simulink model "s_c_nbe_m1k"  (R2016b)
settings: Solver=VariableStepAuto  StartTime=0.0  StopTime=1000  RelTol=1e-3  EnableMultiTasking=on
undefined symbols (not defined in the file): Coeffs, fft_stages, n_taps, output_bits, pfb_coeff_gen_calc, xengbits
libraries: xbsIndex_r4 x23639, casper_library_misc x65, casper_library_scopes x4, xbsReplacements_r4 x4, xps_library x3
(part 36 of 198)

== system s_c_nbe_m1k/DDC/dec_fir_async3 ==
  sync_in : Inport
  dv_in : Inport  Port=2
  real1 : Inport  Port=3
  imag1 : Inport  Port=4
  real2 : Inport  Port=5
  imag2 : Inport  Port=6
  real3 : Inport  Port=7
  imag3 : Inport  Port=8
  real4 : Inport  Port=9
  imag4 : Inport  Port=10
  real5 : Inport  Port=11
  imag5 : Inport  Port=12
  real6 : Inport  Port=13
  imag6 : Inport  Port=14
  real7 : Inport  Port=15
  imag7 : Inport  Port=16
  real8 : Inport  Port=17
  imag8 : Inport  Port=18
  real9 : Inport  Port=19
  imag9 : Inport  Port=20
  real10 : Inport  Port=21
  imag10 : Inport  Port=22
  real11 : Inport  Port=23
  imag11 : Inport  Port=24
  real12 : Inport  Port=25
  imag12 : Inport  Port=26
  real13 : Inport  Port=27
  imag13 : Inport  Port=28
  real14 : Inport  Port=29
  imag14 : Inport  Port=30
  real15 : Inport  Port=31
  imag15 : Inport  Port=32
  real16 : Inport  Port=33
  imag16 : Inport  Port=34
  Logical : xbsIndex_r4/Logical  logical_function=OR  inputs=2  en=off  latency=0  precision=Full  arith_type=Unsigned  n_bits=16  bin_pt=0  align_bp=on  dbl_ovrd=off  block_type=logical
  convert_of : Subsystem  AncestorBlock=casper_library_misc/convert_of  mask(convert_of){bit_width_i=44, binary_point_i=34, bit_width_o=18, binary_point_o=17, latency=2, overflow=Saturate, quantization=Round  (unbiased: +/- Inf)}
      mask prompts: bit_width_i "Bit Width In"; binary_point_i "Binary Point In"; bit_width_o "Bit Width Out"; binary_point_o "Binary Point Out"; overflow "Overflow Behaviour"; quantization "Quantization Behaviour"
      mask help:
      | Converts from one 2's complement bit-width
      | and/or binary point position to another.
      | Includes underflow/overflow indicator.
      mask init: same as s_c_nbe_m1k/DDC/dec_fir_async2/convert_of
      settings: AttributesFormatString=[44,34]->[18,17]
      mask TypeOptions overflow: Wrap | Saturate | Error
      mask TypeOptions quantization: Truncate | Round  (unbiased: +/- Inf) | Round  (unbiased: even values)
  convert_of1 : Subsystem  AncestorBlock=casper_library_misc/convert_of  mask(convert_of){bit_width_i=44, binary_point_i=34, bit_width_o=18, binary_point_o=17, latency=2, overflow=Saturate, quantization=Round  (unbiased: +/- Inf)}
      mask prompts: bit_width_i "Bit Width In"; binary_point_i "Binary Point In"; bit_width_o "Bit Width Out"; binary_point_o "Binary Point Out"; overflow "Overflow Behaviour"; quantization "Quantization Behaviour"
      mask help:
      | Converts from one 2's complement bit-width
      | and/or binary point position to another.
      | Includes underflow/overflow indicator.
      mask init: same as s_c_nbe_m1k/DDC/dec_fir_async2/convert_of
      settings: AttributesFormatString=[44,34]->[18,17]
      mask TypeOptions overflow: Wrap | Saturate | Error
      mask TypeOptions quantization: Truncate | Round  (unbiased: +/- Inf) | Round  (unbiased: even values)
  dv_delay : xbsIndex_r4/Delay  rst=off  infoeditControl=Selection of Reset will increase slice count due to use of real FFs and instead of SRLs  en=off  latency=70  reg_retiming=off  dbl_ovrd=off  block_type=delay
      settings: infoedit=Hardware notes: A delay line is a chain, each link of which is an SRL16 or SRL32 followed by a flip-flop.
  fir_col_async1 : Subsystem  AncestorBlock=casper_library_downconverter/fir_col_async  mask(fir_col_async){n_inputs=16, coeff=[-0.0014387  -0.0013164  -0.0011904  -0.0010635 -0.00093843 -0.00081728 -0.00070197   -0.000594 -0.00049456 -0.00040436 -0.00032436 -0.00025272 -0.00019764 -0.00012413  -0.0001761 -3.7164e-05], add_latency=7, mult_latency=7, coeff_bit_width=18, coeff_bin_pt=17, first_stage_hdl=on, adder_imp=DSP48, async=on, bus_input=off, input_width=0, input_bp=0, input_type=Signed, dbl=on}
      mask prompts: n_inputs "Inputs"; coeff "Coefficients"; add_latency "Add latency"; mult_latency "Mult Latency"; coeff_bit_width "Coefficient bit width"; coeff_bin_pt "Coefficient binary point"; first_stage_hdl "Implement first stage of adder trees on output as behavioural HDL"; adder_imp "Adder implementation"; async "Asynchronous ops"; bus_input "Bus input"; input_width "Input bitwidth"; input_bp "Input binary point"; input_type "Input datatype"; dbl "Double col"
      mask init:
      | fir_col_async_init(gcb);
      mask Help: eval('xlWeb(''http://casper.berkeley.edu/wiki/Fir_col'')')
      mask TypeOptions adder_imp: Behavioral | Fabric | DSP48
      mask Callback bus_input:
      | onoff = get_param(gcb, 'bus_input');
      | set_param_state(gcb, 'input_width', onoff)
      | set_param_state(gcb, 'input_bp', onoff)
      | set_param_state(gcb, 'input_type', onoff)
      mask TypeOptions input_type: Signed | Unsigned
  fir_col_async2 : Subsystem  AncestorBlock=casper_library_downconverter/fir_col_async  mask(fir_col_async){n_inputs=16, coeff=[-0.00060248  -0.0008629  -0.0011001  -0.0013106  -0.0014916  -0.0016412  -0.0017585  -0.0018435  -0.0018966  -0.0019194  -0.0019136  -0.0018817  -0.0018267  -0.0017515  -0.0016595  -0.0015541], add_latency=7, mult_latency=7, coeff_bit_width=18, coeff_bin_pt=17, first_stage_hdl=on, adder_imp=DSP48, async=on, bus_input=off, input_width=0, input_bp=0, input_type=Signed, dbl=on}
      mask prompts: n_inputs "Inputs"; coeff "Coefficients"; add_latency "Add latency"; mult_latency "Mult Latency"; coeff_bit_width "Coefficient bit width"; coeff_bin_pt "Coefficient binary point"; first_stage_hdl "Implement first stage of adder trees on output as behavioural HDL"; adder_imp "Adder implementation"; async "Asynchronous ops"; bus_input "Bus input"; input_width "Input bitwidth"; input_bp "Input binary point"; input_type "Input datatype"; dbl "Double col"
      mask init:
      | fir_col_async_init(gcb);
      mask Help: eval('xlWeb(''http://casper.berkeley.edu/wiki/Fir_col'')')
      mask TypeOptions adder_imp: Behavioral | Fabric | DSP48
      mask Callback bus_input:
      | onoff = get_param(gcb, 'bus_input');
      | set_param_state(gcb, 'input_width', onoff)
      | set_param_state(gcb, 'input_bp', onoff)
      | set_param_state(gcb, 'input_type', onoff)
      mask TypeOptions input_type: Signed | Unsigned
  fir_col_async3 : Subsystem  AncestorBlock=casper_library_downconverter/fir_col_async  mask(fir_col_async){n_inputs=16, coeff=[0.0017612   0.0019473    0.002073   0.0021379   0.0021431   0.0020913   0.0019861   0.0018327    0.001637   0.0014057   0.0011457  0.00086469  0.00057007  0.00026925 -3.0764e-05 -0.00032335], add_latency=7, mult_latency=7, coeff_bit_width=18, coeff_bin_pt=17, first_stage_hdl=on, adder_imp=DSP48, async=on, bus_input=off, input_width=0, input_bp=0, input_type=Signed, dbl=on}
      mask prompts: n_inputs "Inputs"; coeff "Coefficients"; add_latency "Add latency"; mult_latency "Mult Latency"; coeff_bit_width "Coefficient bit width"; coeff_bin_pt "Coefficient binary point"; first_stage_hdl "Implement first stage of adder trees on output as behavioural HDL"; adder_imp "Adder implementation"; async "Asynchronous ops"; bus_input "Bus input"; input_width "Input bitwidth"; input_bp "Input binary point"; input_type "Input datatype"; dbl "Double col"
      mask init:
      | fir_col_async_init(gcb);
      mask Help: eval('xlWeb(''http://casper.berkeley.edu/wiki/Fir_col'')')
      mask TypeOptions adder_imp: Behavioral | Fabric | DSP48
      mask Callback bus_input:
      | onoff = get_param(gcb, 'bus_input');
      | set_param_state(gcb, 'input_width', onoff)
      | set_param_state(gcb, 'input_bp', onoff)
      | set_param_state(gcb, 'input_type', onoff)
      mask TypeOptions input_type: Signed | Unsigned
  fir_col_async4 : Subsystem  AncestorBlock=casper_library_downconverter/fir_col_async  mask(fir_col_async){n_inputs=16, coeff=[-0.0034012  -0.0033949  -0.0032965  -0.0031135   -0.002855  -0.0025319  -0.0021562  -0.0017405  -0.0012982 -0.00084229  -0.0003857  5.9318e-05  0.00048145  0.00087067   0.0012182   0.0015169], add_latency=7, mult_latency=7, coeff_bit_width=18, coeff_bin_pt=17, first_stage_hdl=on, adder_imp=DSP48, async=on, bus_input=off, input_width=0, input_bp=0, input_type=Signed, dbl=on}
      mask prompts: n_inputs "Inputs"; coeff "Coefficients"; add_latency "Add latency"; mult_latency "Mult Latency"; coeff_bit_width "Coefficient bit width"; coeff_bin_pt "Coefficient binary point"; first_stage_hdl "Implement first stage of adder trees on output as behavioural HDL"; adder_imp "Adder implementation"; async "Asynchronous ops"; bus_input "Bus input"; input_width "Input bitwidth"; input_bp "Input binary point"; input_type "Input datatype"; dbl "Double col"
      mask init:
      | fir_col_async_init(gcb);
      mask Help: eval('xlWeb(''http://casper.berkeley.edu/wiki/Fir_col'')')
      mask TypeOptions adder_imp: Behavioral | Fabric | DSP48
      mask Callback bus_input:
      | onoff = get_param(gcb, 'bus_input');
      | set_param_state(gcb, 'input_width', onoff)
      | set_param_state(gcb, 'input_bp', onoff)
      | set_param_state(gcb, 'input_type', onoff)
      mask TypeOptions input_type: Signed | Unsigned
  fir_col_async5 : Subsystem  AncestorBlock=casper_library_downconverter/fir_col_async  mask(fir_col_async){n_inputs=16, coeff=[0.0052142   0.0047761   0.0042315    0.003601   0.0029062   0.0021698   0.0014136  0.00065938 -7.2712e-05 -0.00076401  -0.0013979  -0.0019605  -0.0024401  -0.0028283  -0.0031192  -0.0033102], add_latency=7, mult_latency=7, coeff_bit_width=18, coeff_bin_pt=17, first_stage_hdl=on, adder_imp=DSP48, async=on, bus_input=off, input_width=0, input_bp=0, input_type=Signed, dbl=on}
      mask prompts: n_inputs "Inputs"; coeff "Coefficients"; add_latency "Add latency"; mult_latency "Mult Latency"; coeff_bit_width "Coefficient bit width"; coeff_bin_pt "Coefficient binary point"; first_stage_hdl "Implement first stage of adder trees on output as behavioural HDL"; adder_imp "Adder implementation"; async "Asynchronous ops"; bus_input "Bus input"; input_width "Input bitwidth"; input_bp "Input binary point"; input_type "Input datatype"; dbl "Double col"
      mask init:
      | fir_col_async_init(gcb);
      mask Help: eval('xlWeb(''http://casper.berkeley.edu/wiki/Fir_col'')')
      mask TypeOptions adder_imp: Behavioral | Fabric | DSP48
      mask Callback bus_input:
      | onoff = get_param(gcb, 'bus_input');
      | set_param_state(gcb, 'input_width', onoff)
      | set_param_state(gcb, 'input_bp', onoff)
      | set_param_state(gcb, 'input_type', onoff)
      mask TypeOptions input_type: Signed | Unsigned
  fir_col_async6 : Subsystem  AncestorBlock=casper_library_downconverter/fir_col_async  mask(fir_col_async){n_inputs=16, coeff=[-0.0066831  -0.0053985  -0.0040541  -0.0026891  -0.0013407 -4.3146e-05   0.0011726   0.0022795   0.0032551   0.0040817   0.0047463   0.0052409   0.0055625   0.0057127   0.0056974   0.0055268], add_latency=7, mult_latency=7, coeff_bit_width=18, coeff_bin_pt=17, first_stage_hdl=on, adder_imp=DSP48, async=on, bus_input=off, input_width=0, input_bp=0, input_type=Signed, dbl=on}
      mask prompts: n_inputs "Inputs"; coeff "Coefficients"; add_latency "Add latency"; mult_latency "Mult Latency"; coeff_bit_width "Coefficient bit width"; coeff_bin_pt "Coefficient binary point"; first_stage_hdl "Implement first stage of adder trees on output as behavioural HDL"; adder_imp "Adder implementation"; async "Asynchronous ops"; bus_input "Bus input"; input_width "Input bitwidth"; input_bp "Input binary point"; input_type "Input datatype"; dbl "Double col"
      mask init:
      | fir_col_async_init(gcb);
      mask Help: eval('xlWeb(''http://casper.berkeley.edu/wiki/Fir_col'')')
      mask TypeOptions adder_imp: Behavioral | Fabric | DSP48
      mask Callback bus_input:
      | onoff = get_param(gcb, 'bus_input');
      | set_param_state(gcb, 'input_width', onoff)
      | set_param_state(gcb, 'input_bp', onoff)
      | set_param_state(gcb, 'input_type', onoff)
      mask TypeOptions input_type: Signed | Unsigned
  fir_col_async7 : Subsystem  AncestorBlock=casper_library_downconverter/fir_col_async  mask(fir_col_async){n_inputs=16, coeff=[0.0069344   0.0036796   0.0006949  -0.0019856   -0.004335  -0.0063338  -0.0079699   -0.009239   -0.010144   -0.010695   -0.010908   -0.010806   -0.010418   -0.009774  -0.0089111  -0.0078675], add_latency=7, mult_latency=7, coeff_bit_width=18, coeff_bin_pt=17, first_stage_hdl=on, adder_imp=DSP48, async=on, bus_input=off, input_width=0, input_bp=0, input_type=Signed, dbl=on}
      mask prompts: n_inputs "Inputs"; coeff "Coefficients"; add_latency "Add latency"; mult_latency "Mult Latency"; coeff_bit_width "Coefficient bit width"; coeff_bin_pt "Coefficient binary point"; first_stage_hdl "Implement first stage of adder trees on output as behavioural HDL"; adder_imp "Adder implementation"; async "Asynchronous ops"; bus_input "Bus input"; input_width "Input bitwidth"; input_bp "Input binary point"; input_type "Input datatype"; dbl "Double col"
      mask init:
      | fir_col_async_init(gcb);
      mask Help: eval('xlWeb(''http://casper.berkeley.edu/wiki/Fir_col'')')
      mask TypeOptions adder_imp: Behavioral | Fabric | DSP48
      mask Callback bus_input:
      | onoff = get_param(gcb, 'bus_input');
      | set_param_state(gcb, 'input_width', onoff)
      | set_param_state(gcb, 'input_bp', onoff)
      | set_param_state(gcb, 'input_type', onoff)
      mask TypeOptions input_type: Signed | Unsigned
  fir_col_async8 : Subsystem  AncestorBlock=casper_library_downconverter/fir_col_async  mask(fir_col_async){n_inputs=16, coeff=[0.053294    0.052787    0.051782    0.050297    0.048358    0.045997    0.043256    0.040183    0.036828    0.033249    0.029504    0.025654    0.021761    0.017886    0.014086    0.010419], add_latency=7, mult_latency=7, coeff_bit_width=18, coeff_bin_pt=17, first_stage_hdl=on, adder_imp=DSP48, async=on, bus_input=off, input_width=0, input_bp=0, input_type=Signed, dbl=on}
      mask prompts: n_inputs "Inputs"; coeff "Coefficients"; add_latency "Add latency"; mult_latency "Mult Latency"; coeff_bit_width "Coefficient bit width"; coeff_bin_pt "Coefficient binary point"; first_stage_hdl "Implement first stage of adder trees on output as behavioural HDL"; adder_imp "Adder implementation"; async "Asynchronous ops"; bus_input "Bus input"; input_width "Input bitwidth"; input_bp "Input binary point"; input_type "Input datatype"; dbl "Double col"
      mask init:
      | fir_col_async_init(gcb);
      mask Help: eval('xlWeb(''http://casper.berkeley.edu/wiki/Fir_col'')')
      mask TypeOptions adder_imp: Behavioral | Fabric | DSP48
      mask Callback bus_input:
      | onoff = get_param(gcb, 'bus_input');
      | set_param_state(gcb, 'input_width', onoff)
      | set_param_state(gcb, 'input_bp', onoff)
      | set_param_state(gcb, 'input_type', onoff)
      mask TypeOptions input_type: Signed | Unsigned
  imag_sum : Subsystem  AncestorBlock=casper_library_misc/adder_tree  mask(adder_tree){n_inputs=8, latency=7, adder_imp=DSP48, first_stage_hdl=off, floating_point=off, float_type=single, frac_width=0, exp_width=0}
      mask prompts: n_inputs "Number of Inputs"; latency "Add Latency"; adder_imp "Adder implementation"; first_stage_hdl "Use behavioural HDL for first stage of adders"; floating_point "floating point"; float_type "float type"; frac_width "fraction length"; exp_width "exponent length"
      mask help:
      | Sums all inputs using a tree of adds and delays.
      |
      | Number of inputs: The number of inputs to the block to be summed
      | Add latency: The number of clock cycles to perform one addition (affects timing)..
      | Adder implementation: choice of fabric or DSP48E core, or behavioral HDL
      | Use behavioural HDL for first stage of adders: Causes the first stage of adders to be absorbed into DSP blocks if multipliers precede them (Virtex 5). Overrides Adder implementation
      mask init: same as s_c_nbe_m1k/DDC/dec_fir_async1/imag_sum
      settings: AttributesFormatString=latency 21
      mask Help: eval('xlWeb(''http://casper.berkeley.edu/wiki/Adder_tree'')')
      mask TypeOptions adder_imp: Behavioral | Fabric | DSP48
      mask Callback floating_point:
      | onoff = get_param(gcb, 'floating_point');
      | if strcmp(onoff,'on')
      |     enable_fixpt = 'off'
      |     set_param_state(gcb, 'float_type', 'on')
      | 
      |     f_type = get_param(gcb, 'float_type')
      |     if strcmp(f_type,'custom')
      |         set_param_state(gcb, 'exp_width', 'on')
      |         set_param_state(gcb, 'frac_width', 'on')
      |     else
      |         set_param_state(gcb, 'exp_width', 'off')
      |         set_param_state(gcb, 'frac_width', 'off')
      |     end
      | 
      | 
      | else
      |     enable_fixpt = 'on'
      |     set_param_state(gcb, 'float_type', 'off')
      |     set_param_state(gcb, 'exp_width', 'off')
      |     set_param_state(gcb, 'frac_width', 'off')
      | end
      mask TypeOptions float_type: single | custom
      mask Callback float_type:
      | f_type = get_param(gcb, 'float_type')
      | if strcmp(f_type,'custom')
      |     set_param_state(gcb, 'exp_width', 'on')
      |     set_param_state(gcb, 'frac_width', 'on')
      | else
      |     set_param_state(gcb, 'exp_width', 'off')
      |     set_param_state(gcb, 'frac_width', 'off')
      | end
  real_sum : Subsystem  AncestorBlock=casper_library_misc/adder_tree  mask(adder_tree){n_inputs=8, latency=7, adder_imp=DSP48, first_stage_hdl=off, floating_point=off, float_type=single, frac_width=0, exp_width=0}
      mask prompts: n_inputs "Number of Inputs"; latency "Add Latency"; adder_imp "Adder implementation"; first_stage_hdl "Use behavioural HDL for first stage of adders"; floating_point "floating point"; float_type "float type"; frac_width "fraction length"; exp_width "exponent length"
      mask help:
      | Sums all inputs using a tree of adds and delays.
      |
      | Number of inputs: The number of inputs to the block to be summed
      | Add latency: The number of clock cycles to perform one addition (affects timing)..
      | Adder implementation: choice of fabric or DSP48E core, or behavioral HDL
      | Use behavioural HDL for first stage of adders: Causes the first stage of adders to be absorbed into DSP blocks if multipliers precede them (Virtex 5). Overrides Adder implementation
      mask init: same as s_c_nbe_m1k/DDC/dec_fir_async1/imag_sum
      settings: AttributesFormatString=latency 21
      mask Help: eval('xlWeb(''http://casper.berkeley.edu/wiki/Adder_tree'')')
      mask TypeOptions adder_imp: Behavioral | Fabric | DSP48
      mask Callback floating_point:
      | onoff = get_param(gcb, 'floating_point');
      | if strcmp(onoff,'on')
      |     enable_fixpt = 'off'
      |     set_param_state(gcb, 'float_type', 'on')
      | 
      |     f_type = get_param(gcb, 'float_type')
      |     if strcmp(f_type,'custom')
      |         set_param_state(gcb, 'exp_width', 'on')
      |         set_param_state(gcb, 'frac_width', 'on')
      |     else
      |         set_param_state(gcb, 'exp_width', 'off')
      |         set_param_state(gcb, 'frac_width', 'off')
      |     end
      | 
      | 
      | else
      |     enable_fixpt = 'on'
      |     set_param_state(gcb, 'float_type', 'off')
      |     set_param_state(gcb, 'exp_width', 'off')
      |     set_param_state(gcb, 'frac_width', 'off')
      | end
      mask TypeOptions float_type: single | custom
      mask Callback float_type:
      | f_type = get_param(gcb, 'float_type')
      | if strcmp(f_type,'custom')
      |     set_param_state(gcb, 'exp_width', 'on')
      |     set_param_state(gcb, 'frac_width', 'on')
      | else
      |     set_param_state(gcb, 'exp_width', 'off')
      |     set_param_state(gcb, 'frac_width', 'off')
      | end
  ri_to_c1 : casper_library_misc/ri_to_c
  shift1 : xbsIndex_r4/Shift  shift_dir=Left  shift_bits=1  en=off  latency=1  precision=Full  arith_type="Signed  (2's comp)"  n_bits=16  bin_pt=14  quantization=Truncate  overflow=Wrap  dbl_ovrd=off  block_type=shift
  shift2 : xbsIndex_r4/Shift  shift_dir=Left  shift_bits=1  en=off  latency=1  precision=Full  arith_type="Signed  (2's comp)"  n_bits=16  bin_pt=14  quantization=Truncate  overflow=Wrap  dbl_ovrd=off  block_type=shift
  sync_delay : xbsIndex_r4/Delay  rst=off  infoeditControl=Selection of Reset will increase slice count due to use of real FFs and instead of SRLs  en=off  latency=49  reg_retiming=off  dbl_ovrd=off  block_type=delay
      settings: infoedit=Hardware notes: A delay line is a chain, each link of which is an SRL16 or SRL32 followed by a flip-flop.
  sync_out : Outport
  dout : Outport  Port=2
  dv_out : Outport  Port=3
  of : Outport  Port=4
  wires:
  Logical/1 -> of/1
  ri_to_c1/1 -> dout/1
  convert_of1/1(dout) -> ri_to_c1/2
  convert_of/1(dout) -> ri_to_c1/1
  convert_of/2(of) -> Logical/1
  convert_of1/2(of) -> Logical/2
  fir_col_async8/32(imag_out16) -> fir_col_async8/64(imag_back16)
  fir_col_async8/31(real_out16) -> fir_col_async8/63(real_back16)
  fir_col_async8/30(imag_out15) -> fir_col_async8/62(imag_back15)
  fir_col_async8/29(real_out15) -> fir_col_async8/61(real_back15)
  fir_col_async8/28(imag_out14) -> fir_col_async8/60(imag_back14)
  fir_col_async8/27(real_out14) -> fir_col_async8/59(real_back14)
  fir_col_async8/26(imag_out13) -> fir_col_async8/58(imag_back13)
  fir_col_async8/25(real_out13) -> fir_col_async8/57(real_back13)
  fir_col_async8/24(imag_out12) -> fir_col_async8/56(imag_back12)
  fir_col_async8/23(real_out12) -> fir_col_async8/55(real_back12)
  fir_col_async8/22(imag_out11) -> fir_col_async8/54(imag_back11)
  fir_col_async8/21(real_out11) -> fir_col_async8/53(real_back11)
  fir_col_async8/20(imag_out10) -> fir_col_async8/52(imag_back10)
  fir_col_async8/19(real_out10) -> fir_col_async8/51(real_back10)
  fir_col_async8/18(imag_out9) -> fir_col_async8/50(imag_back9)
  fir_col_async8/17(real_out9) -> fir_col_async8/49(real_back9)
  fir_col_async8/16(imag_out8) -> fir_col_async8/48(imag_back8)
  fir_col_async8/15(real_out8) -> fir_col_async8/47(real_back8)
  fir_col_async8/14(imag_out7) -> fir_col_async8/46(imag_back7)
  fir_col_async8/13(real_out7) -> fir_col_async8/45(real_back7)
  fir_col_async8/12(imag_out6) -> fir_col_async8/44(imag_back6)
  fir_col_async8/11(real_out6) -> fir_col_async8/43(real_back6)
  fir_col_async8/10(imag_out5) -> fir_col_async8/42(imag_back5)
  fir_col_async8/9(real_out5) -> fir_col_async8/41(real_back5)
  fir_col_async8/8(imag_out4) -> fir_col_async8/40(imag_back4)
  fir_col_async8/7(real_out4) -> fir_col_async8/39(real_back4)
  fir_col_async8/6(imag_out3) -> fir_col_async8/38(imag_back3)
  fir_col_async8/5(real_out3) -> fir_col_async8/37(real_back3)
  fir_col_async8/4(imag_out2) -> fir_col_async8/36(imag_back2)
  fir_col_async8/3(real_out2) -> fir_col_async8/35(real_back2)
  fir_col_async8/2(imag_out1) -> fir_col_async8/34(imag_back1)
  fir_col_async8/1(real_out1) -> fir_col_async8/33(real_back1)
  fir_col_async8/64(imag_back_out16) -> fir_col_async7/64(imag_back16)
  fir_col_async8/63(real_back_out16) -> fir_col_async7/63(real_back16)
  fir_col_async8/62(imag_back_out15) -> fir_col_async7/62(imag_back15)
  fir_col_async8/61(real_back_out15) -> fir_col_async7/61(real_back15)
  fir_col_async8/60(imag_back_out14) -> fir_col_async7/60(imag_back14)
  fir_col_async8/59(real_back_out14) -> fir_col_async7/59(real_back14)
  fir_col_async8/58(imag_back_out13) -> fir_col_async7/58(imag_back13)
  fir_col_async8/57(real_back_out13) -> fir_col_async7/57(real_back13)
  fir_col_async8/56(imag_back_out12) -> fir_col_async7/56(imag_back12)
  fir_col_async8/55(real_back_out12) -> fir_col_async7/55(real_back12)
  fir_col_async8/54(imag_back_out11) -> fir_col_async7/54(imag_back11)
  fir_col_async8/53(real_back_out11) -> fir_col_async7/53(real_back11)
  fir_col_async8/52(imag_back_out10) -> fir_col_async7/52(imag_back10)
  fir_col_async8/51(real_back_out10) -> fir_col_async7/51(real_back10)
  fir_col_async8/50(imag_back_out9) -> fir_col_async7/50(imag_back9)
  fir_col_async8/49(real_back_out9) -> fir_col_async7/49(real_back9)
  fir_col_async8/48(imag_back_out8) -> fir_col_async7/48(imag_back8)
  fir_col_async8/47(real_back_out8) -> fir_col_async7/47(real_back8)
  fir_col_async8/46(imag_back_out7) -> fir_col_async7/46(imag_back7)
  fir_col_async8/45(real_back_out7) -> fir_col_async7/45(real_back7)
  fir_col_async8/44(imag_back_out6) -> fir_col_async7/44(imag_back6)
  fir_col_async8/43(real_back_out6) -> fir_col_async7/43(real_back6)
  fir_col_async8/42(imag_back_out5) -> fir_col_async7/42(imag_back5)
  fir_col_async8/41(real_back_out5) -> fir_col_async7/41(real_back5)
  fir_col_async8/40(imag_back_out4) -> fir_col_async7/40(imag_back4)
  fir_col_async8/39(real_back_out4) -> fir_col_async7/39(real_back4)
  fir_col_async8/38(imag_back_out3) -> fir_col_async7/38(imag_back3)
  fir_col_async8/37(real_back_out3) -> fir_col_async7/37(real_back3)
  fir_col_async8/36(imag_back_out2) -> fir_col_async7/36(imag_back2)
  fir_col_async8/35(real_back_out2) -> fir_col_async7/35(real_back2)
  fir_col_async8/34(imag_back_out1) -> fir_col_async7/34(imag_back1)
  fir_col_async8/33(real_back_out1) -> fir_col_async7/33(real_back1)
  fir_col_async7/64(imag_back_out16) -> fir_col_async6/64(imag_back16)
  fir_col_async7/63(real_back_out16) -> fir_col_async6/63(real_back16)
  fir_col_async7/62(imag_back_out15) -> fir_col_async6/62(imag_back15)
  fir_col_async7/61(real_back_out15) -> fir_col_async6/61(real_back15)
  fir_col_async7/60(imag_back_out14) -> fir_col_async6/60(imag_back14)
  fir_col_async7/59(real_back_out14) -> fir_col_async6/59(real_back14)
  fir_col_async7/58(imag_back_out13) -> fir_col_async6/58(imag_back13)
  fir_col_async7/57(real_back_out13) -> fir_col_async6/57(real_back13)
  fir_col_async7/56(imag_back_out12) -> fir_col_async6/56(imag_back12)
  fir_col_async7/55(real_back_out12) -> fir_col_async6/55(real_back12)
  fir_col_async7/54(imag_back_out11) -> fir_col_async6/54(imag_back11)
  fir_col_async7/53(real_back_out11) -> fir_col_async6/53(real_back11)
  fir_col_async7/52(imag_back_out10) -> fir_col_async6/52(imag_back10)
  fir_col_async7/51(real_back_out10) -> fir_col_async6/51(real_back10)
  fir_col_async7/50(imag_back_out9) -> fir_col_async6/50(imag_back9)
  fir_col_async7/49(real_back_out9) -> fir_col_async6/49(real_back9)
  fir_col_async7/48(imag_back_out8) -> fir_col_async6/48(imag_back8)
  fir_col_async7/47(real_back_out8) -> fir_col_async6/47(real_back8)
  fir_col_async7/46(imag_back_out7) -> fir_col_async6/46(imag_back7)
  fir_col_async7/45(real_back_out7) -> fir_col_async6/45(real_back7)
  fir_col_async7/44(imag_back_out6) -> fir_col_async6/44(imag_back6)
  fir_col_async7/43(real_back_out6) -> fir_col_async6/43(real_back6)
  fir_col_async7/42(imag_back_out5) -> fir_col_async6/42(imag_back5)
  fir_col_async7/41(real_back_out5) -> fir_col_async6/41(real_back5)
  fir_col_async7/40(imag_back_out4) -> fir_col_async6/40(imag_back4)
  fir_col_async7/39(real_back_out4) -> fir_col_async6/39(real_back4)
  fir_col_async7/38(imag_back_out3) -> fir_col_async6/38(imag_back3)
  fir_col_async7/37(real_back_out3) -> fir_col_async6/37(real_back3)
  fir_col_async7/36(imag_back_out2) -> fir_col_async6/36(imag_back2)
  fir_col_async7/35(real_back_out2) -> fir_col_async6/35(real_back2)
  fir_col_async7/34(imag_back_out1) -> fir_col_async6/34(imag_back1)
  fir_col_async7/33(real_back_out1) -> fir_col_async6/33(real_back1)
  fir_col_async6/64(imag_back_out16) -> fir_col_async5/64(imag_back16)
  fir_col_async6/63(real_back_out16) -> fir_col_async5/63(real_back16)
  fir_col_async6/62(imag_back_out15) -> fir_col_async5/62(imag_back15)
  fir_col_async6/61(real_back_out15) -> fir_col_async5/61(real_back15)
  fir_col_async6/60(imag_back_out14) -> fir_col_async5/60(imag_back14)
  fir_col_async6/59(real_back_out14) -> fir_col_async5/59(real_back14)
  fir_col_async6/58(imag_back_out13) -> fir_col_async5/58(imag_back13)
  fir_col_async6/57(real_back_out13) -> fir_col_async5/57(real_back13)
  fir_col_async6/56(imag_back_out12) -> fir_col_async5/56(imag_back12)
  fir_col_async6/55(real_back_out12) -> fir_col_async5/55(real_back12)
  fir_col_async6/54(imag_back_out11) -> fir_col_async5/54(imag_back11)
  fir_col_async6/53(real_back_out11) -> fir_col_async5/53(real_back11)
  fir_col_async6/52(imag_back_out10) -> fir_col_async5/52(imag_back10)
  fir_col_async6/51(real_back_out10) -> fir_col_async5/51(real_back10)
  fir_col_async6/50(imag_back_out9) -> fir_col_async5/50(imag_back9)
  fir_col_async6/49(real_back_out9) -> fir_col_async5/49(real_back9)
  fir_col_async6/48(imag_back_out8) -> fir_col_async5/48(imag_back8)
  fir_col_async6/47(real_back_out8) -> fir_col_async5/47(real_back8)
  fir_col_async6/46(imag_back_out7) -> fir_col_async5/46(imag_back7)
  fir_col_async6/45(real_back_out7) -> fir_col_async5/45(real_back7)
  fir_col_async6/44(imag_back_out6) -> fir_col_async5/44(imag_back6)
  fir_col_async6/43(real_back_out6) -> fir_col_async5/43(real_back6)
  fir_col_async6/42(imag_back_out5) -> fir_col_async5/42(imag_back5)
  fir_col_async6/41(real_back_out5) -> fir_col_async5/41(real_back5)
  fir_col_async6/40(imag_back_out4) -> fir_col_async5/40(imag_back4)
  fir_col_async6/39(real_back_out4) -> fir_col_async5/39(real_back4)
  fir_col_async6/38(imag_back_out3) -> fir_col_async5/38(imag_back3)
  fir_col_async6/37(real_back_out3) -> fir_col_async5/37(real_back3)
  fir_col_async6/36(imag_back_out2) -> fir_col_async5/36(imag_back2)
  fir_col_async6/35(real_back_out2) -> fir_col_async5/35(real_back2)
  fir_col_async6/34(imag_back_out1) -> fir_col_async5/34(imag_back1)
  fir_col_async6/33(real_back_out1) -> fir_col_async5/33(real_back1)
  fir_col_async5/64(imag_back_out16) -> fir_col_async4/64(imag_back16)
  fir_col_async5/63(real_back_out16) -> fir_col_async4/63(real_back16)
  fir_col_async5/62(imag_back_out15) -> fir_col_async4/62(imag_back15)
  fir_col_async5/61(real_back_out15) -> fir_col_async4/61(real_back15)
  fir_col_async5/60(imag_back_out14) -> fir_col_async4/60(imag_back14)
  fir_col_async5/59(real_back_out14) -> fir_col_async4/59(real_back14)
  fir_col_async5/58(imag_back_out13) -> fir_col_async4/58(imag_back13)
  fir_col_async5/57(real_back_out13) -> fir_col_async4/57(real_back13)
  fir_col_async5/56(imag_back_out12) -> fir_col_async4/56(imag_back12)
  fir_col_async5/55(real_back_out12) -> fir_col_async4/55(real_back12)
  fir_col_async5/54(imag_back_out11) -> fir_col_async4/54(imag_back11)
  fir_col_async5/53(real_back_out11) -> fir_col_async4/53(real_back11)
  fir_col_async5/52(imag_back_out10) -> fir_col_async4/52(imag_back10)
  fir_col_async5/51(real_back_out10) -> fir_col_async4/51(real_back10)
  fir_col_async5/50(imag_back_out9) -> fir_col_async4/50(imag_back9)
  fir_col_async5/49(real_back_out9) -> fir_col_async4/49(real_back9)
  fir_col_async5/48(imag_back_out8) -> fir_col_async4/48(imag_back8)
  fir_col_async5/47(real_back_out8) -> fir_col_async4/47(real_back8)
  fir_col_async5/46(imag_back_out7) -> fir_col_async4/46(imag_back7)
  fir_col_async5/45(real_back_out7) -> fir_col_async4/45(real_back7)
  fir_col_async5/44(imag_back_out6) -> fir_col_async4/44(imag_back6)
  fir_col_async5/43(real_back_out6) -> fir_col_async4/43(real_back6)
  fir_col_async5/42(imag_back_out5) -> fir_col_async4/42(imag_back5)
  fir_col_async5/41(real_back_out5) -> fir_col_async4/41(real_back5)
  fir_col_async5/40(imag_back_out4) -> fir_col_async4/40(imag_back4)
  fir_col_async5/39(real_back_out4) -> fir_col_async4/39(real_back4)
  fir_col_async5/38(imag_back_out3) -> fir_col_async4/38(imag_back3)
  fir_col_async5/37(real_back_out3) -> fir_col_async4/37(real_back3)
  fir_col_async5/36(imag_back_out2) -> fir_col_async4/36(imag_back2)
  fir_col_async5/35(real_back_out2) -> fir_col_async4/35(real_back2)
  fir_col_async5/34(imag_back_out1) -> fir_col_async4/34(imag_back1)
  fir_col_async5/33(real_back_out1) -> fir_col_async4/33(real_back1)
  fir_col_async4/64(imag_back_out16) -> fir_col_async3/64(imag_back16)
  fir_col_async4/63(real_back_out16) -> fir_col_async3/63(real_back16)
  fir_col_async4/62(imag_back_out15) -> fir_col_async3/62(imag_back15)
  fir_col_async4/61(real_back_out15) -> fir_col_async3/61(real_back15)
  fir_col_async4/60(imag_back_out14) -> fir_col_async3/60(imag_back14)
  fir_col_async4/59(real_back_out14) -> fir_col_async3/59(real_back14)
  fir_col_async4/58(imag_back_out13) -> fir_col_async3/58(imag_back13)
  fir_col_async4/57(real_back_out13) -> fir_col_async3/57(real_back13)
  fir_col_async4/56(imag_back_out12) -> fir_col_async3/56(imag_back12)
  fir_col_async4/55(real_back_out12) -> fir_col_async3/55(real_back12)
  fir_col_async4/54(imag_back_out11) -> fir_col_async3/54(imag_back11)
  fir_col_async4/53(real_back_out11) -> fir_col_async3/53(real_back11)
  fir_col_async4/52(imag_back_out10) -> fir_col_async3/52(imag_back10)
  fir_col_async4/51(real_back_out10) -> fir_col_async3/51(real_back10)
  fir_col_async4/50(imag_back_out9) -> fir_col_async3/50(imag_back9)
  fir_col_async4/49(real_back_out9) -> fir_col_async3/49(real_back9)
  fir_col_async4/48(imag_back_out8) -> fir_col_async3/48(imag_back8)
  fir_col_async4/47(real_back_out8) -> fir_col_async3/47(real_back8)
  fir_col_async4/46(imag_back_out7) -> fir_col_async3/46(imag_back7)
  fir_col_async4/45(real_back_out7) -> fir_col_async3/45(real_back7)
  fir_col_async4/44(imag_back_out6) -> fir_col_async3/44(imag_back6)
  fir_col_async4/43(real_back_out6) -> fir_col_async3/43(real_back6)
  fir_col_async4/42(imag_back_out5) -> fir_col_async3/42(imag_back5)
  fir_col_async4/41(real_back_out5) -> fir_col_async3/41(real_back5)
  fir_col_async4/40(imag_back_out4) -> fir_col_async3/40(imag_back4)
  fir_col_async4/39(real_back_out4) -> fir_col_async3/39(real_back4)
  fir_col_async4/38(imag_back_out3) -> fir_col_async3/38(imag_back3)
  fir_col_async4/37(real_back_out3) -> fir_col_async3/37(real_back3)
  fir_col_async4/36(imag_back_out2) -> fir_col_async3/36(imag_back2)
  fir_col_async4/35(real_back_out2) -> fir_col_async3/35(real_back2)
  fir_col_async4/34(imag_back_out1) -> fir_col_async3/34(imag_back1)
  fir_col_async4/33(real_back_out1) -> fir_col_async3/33(real_back1)
  fir_col_async3/64(imag_back_out16) -> fir_col_async2/64(imag_back16)
  fir_col_async3/63(real_back_out16) -> fir_col_async2/63(real_back16)
  fir_col_async3/62(imag_back_out15) -> fir_col_async2/62(imag_back15)
  fir_col_async3/61(real_back_out15) -> fir_col_async2/61(real_back15)
  fir_col_async3/60(imag_back_out14) -> fir_col_async2/60(imag_back14)
  fir_col_async3/59(real_back_out14) -> fir_col_async2/59(real_back14)
  fir_col_async3/58(imag_back_out13) -> fir_col_async2/58(imag_back13)
  fir_col_async3/57(real_back_out13) -> fir_col_async2/57(real_back13)
  fir_col_async3/56(imag_back_out12) -> fir_col_async2/56(imag_back12)
  fir_col_async3/55(real_back_out12) -> fir_col_async2/55(real_back12)
  fir_col_async3/54(imag_back_out11) -> fir_col_async2/54(imag_back11)
  fir_col_async3/53(real_back_out11) -> fir_col_async2/53(real_back11)
  fir_col_async3/52(imag_back_out10) -> fir_col_async2/52(imag_back10)
  fir_col_async3/51(real_back_out10) -> fir_col_async2/51(real_back10)
  fir_col_async3/50(imag_back_out9) -> fir_col_async2/50(imag_back9)
  fir_col_async3/49(real_back_out9) -> fir_col_async2/49(real_back9)
  fir_col_async3/48(imag_back_out8) -> fir_col_async2/48(imag_back8)
  fir_col_async3/47(real_back_out8) -> fir_col_async2/47(real_back8)
  fir_col_async3/46(imag_back_out7) -> fir_col_async2/46(imag_back7)
  fir_col_async3/45(real_back_out7) -> fir_col_async2/45(real_back7)
  fir_col_async3/44(imag_back_out6) -> fir_col_async2/44(imag_back6)
  fir_col_async3/43(real_back_out6) -> fir_col_async2/43(real_back6)
  fir_col_async3/42(imag_back_out5) -> fir_col_async2/42(imag_back5)
  fir_col_async3/41(real_back_out5) -> fir_col_async2/41(real_back5)
  fir_col_async3/40(imag_back_out4) -> fir_col_async2/40(imag_back4)
  fir_col_async3/39(real_back_out4) -> fir_col_async2/39(real_back4)
  fir_col_async3/38(imag_back_out3) -> fir_col_async2/38(imag_back3)
  fir_col_async3/37(real_back_out3) -> fir_col_async2/37(real_back3)
  fir_col_async3/36(imag_back_out2) -> fir_col_async2/36(imag_back2)
  fir_col_async3/35(real_back_out2) -> fir_col_async2/35(real_back2)
  fir_col_async3/34(imag_back_out1) -> fir_col_async2/34(imag_back1)
  fir_col_async3/33(real_back_out1) -> fir_col_async2/33(real_back1)
  fir_col_async2/64(imag_back_out16) -> fir_col_async1/64(imag_back16)
  fir_col_async2/63(real_back_out16) -> fir_col_async1/63(real_back16)
  fir_col_async2/62(imag_back_out15) -> fir_col_async1/62(imag_back15)
  fir_col_async2/61(real_back_out15) -> fir_col_async1/61(real_back15)
  fir_col_async2/60(imag_back_out14) -> fir_col_async1/60(imag_back14)
  fir_col_async2/59(real_back_out14) -> fir_col_async1/59(real_back14)
  fir_col_async2/58(imag_back_out13) -> fir_col_async1/58(imag_back13)
  fir_col_async2/57(real_back_out13) -> fir_col_async1/57(real_back13)
  fir_col_async2/56(imag_back_out12) -> fir_col_async1/56(imag_back12)
  fir_col_async2/55(real_back_out12) -> fir_col_async1/55(real_back12)
  fir_col_async2/54(imag_back_out11) -> fir_col_async1/54(imag_back11)
  fir_col_async2/53(real_back_out11) -> fir_col_async1/53(real_back11)
  fir_col_async2/52(imag_back_out10) -> fir_col_async1/52(imag_back10)
  fir_col_async2/51(real_back_out10) -> fir_col_async1/51(real_back10)
  fir_col_async2/50(imag_back_out9) -> fir_col_async1/50(imag_back9)
  fir_col_async2/49(real_back_out9) -> fir_col_async1/49(real_back9)
  fir_col_async2/48(imag_back_out8) -> fir_col_async1/48(imag_back8)
  fir_col_async2/47(real_back_out8) -> fir_col_async1/47(real_back8)
  fir_col_async2/46(imag_back_out7) -> fir_col_async1/46(imag_back7)
  fir_col_async2/45(real_back_out7) -> fir_col_async1/45(real_back7)
  fir_col_async2/44(imag_back_out6) -> fir_col_async1/44(imag_back6)
  fir_col_async2/43(real_back_out6) -> fir_col_async1/43(real_back6)
  fir_col_async2/42(imag_back_out5) -> fir_col_async1/42(imag_back5)
  fir_col_async2/41(real_back_out5) -> fir_col_async1/41(real_back5)
  fir_col_async2/40(imag_back_out4) -> fir_col_async1/40(imag_back4)
  fir_col_async2/39(real_back_out4) -> fir_col_async1/39(real_back4)
  fir_col_async2/38(imag_back_out3) -> fir_col_async1/38(imag_back3)
  fir_col_async2/37(real_back_out3) -> fir_col_async1/37(real_back3)
  fir_col_async2/36(imag_back_out2) -> fir_col_async1/36(imag_back2)
  fir_col_async2/35(real_back_out2) -> fir_col_async1/35(real_back2)
  fir_col_async2/34(imag_back_out1) -> fir_col_async1/34(imag_back1)
  fir_col_async2/33(real_back_out1) -> fir_col_async1/33(real_back1)
  real_sum/1(sync_out) -> sync_out/1
  sync_delay/1 -> imag_sum/1(sync), real_sum/1(sync)
  shift2/1 -> convert_of1/1(din)
  shift1/1 -> convert_of/1(din)
  imag_sum/2(dout) -> shift2/1
  real_sum/2(dout) -> shift1/1
  fir_col_async8/66(imag_sum) -> imag_sum/9(din8)
  fir_col_async8/65(real_sum) -> real_sum/9(din8)
  fir_col_async7/32(imag_out16) -> fir_col_async8/32(imag16)
  fir_col_async7/31(real_out16) -> fir_col_async8/31(real16)
  fir_col_async7/30(imag_out15) -> fir_col_async8/30(imag15)
  fir_col_async7/29(real_out15) -> fir_col_async8/29(real15)
  fir_col_async7/28(imag_out14) -> fir_col_async8/28(imag14)
  fir_col_async7/27(real_out14) -> fir_col_async8/27(real14)
  fir_col_async7/26(imag_out13) -> fir_col_async8/26(imag13)
  fir_col_async7/25(real_out13) -> fir_col_async8/25(real13)
  fir_col_async7/24(imag_out12) -> fir_col_async8/24(imag12)
  fir_col_async7/23(real_out12) -> fir_col_async8/23(real12)
  fir_col_async7/22(imag_out11) -> fir_col_async8/22(imag11)
  fir_col_async7/21(real_out11) -> fir_col_async8/21(real11)
  fir_col_async7/20(imag_out10) -> fir_col_async8/20(imag10)
  fir_col_async7/19(real_out10) -> fir_col_async8/19(real10)
  fir_col_async7/18(imag_out9) -> fir_col_async8/18(imag9)
  fir_col_async7/17(real_out9) -> fir_col_async8/17(real9)
  fir_col_async7/16(imag_out8) -> fir_col_async8/16(imag8)
  fir_col_async7/15(real_out8) -> fir_col_async8/15(real8)
  fir_col_async7/14(imag_out7) -> fir_col_async8/14(imag7)
  fir_col_async7/13(real_out7) -> fir_col_async8/13(real7)
  fir_col_async7/12(imag_out6) -> fir_col_async8/12(imag6)
  fir_col_async7/11(real_out6) -> fir_col_async8/11(real6)
  fir_col_async7/10(imag_out5) -> fir_col_async8/10(imag5)
  fir_col_async7/9(real_out5) -> fir_col_async8/9(real5)
  fir_col_async7/8(imag_out4) -> fir_col_async8/8(imag4)
  fir_col_async7/7(real_out4) -> fir_col_async8/7(real4)
  fir_col_async7/6(imag_out3) -> fir_col_async8/6(imag3)
  fir_col_async7/5(real_out3) -> fir_col_async8/5(real3)
  fir_col_async7/4(imag_out2) -> fir_col_async8/4(imag2)
  fir_col_async7/3(real_out2) -> fir_col_async8/3(real2)
  fir_col_async7/2(imag_out1) -> fir_col_async8/2(imag1)
  fir_col_async7/1(real_out1) -> fir_col_async8/1(real1)
  fir_col_async7/66(imag_sum) -> imag_sum/8(din7)
  fir_col_async7/65(real_sum) -> real_sum/8(din7)
  fir_col_async6/32(imag_out16) -> fir_col_async7/32(imag16)
  fir_col_async6/31(real_out16) -> fir_col_async7/31(real16)
  fir_col_async6/30(imag_out15) -> fir_col_async7/30(imag15)
  fir_col_async6/29(real_out15) -> fir_col_async7/29(real15)
  fir_col_async6/28(imag_out14) -> fir_col_async7/28(imag14)
  fir_col_async6/27(real_out14) -> fir_col_async7/27(real14)
  fir_col_async6/26(imag_out13) -> fir_col_async7/26(imag13)
  fir_col_async6/25(real_out13) -> fir_col_async7/25(real13)
  fir_col_async6/24(imag_out12) -> fir_col_async7/24(imag12)
  fir_col_async6/23(real_out12) -> fir_col_async7/23(real12)
  fir_col_async6/22(imag_out11) -> fir_col_async7/22(imag11)
  fir_col_async6/21(real_out11) -> fir_col_async7/21(real11)
  fir_col_async6/20(imag_out10) -> fir_col_async7/20(imag10)
  fir_col_async6/19(real_out10) -> fir_col_async7/19(real10)
  fir_col_async6/18(imag_out9) -> fir_col_async7/18(imag9)
  fir_col_async6/17(real_out9) -> fir_col_async7/17(real9)
  fir_col_async6/16(imag_out8) -> fir_col_async7/16(imag8)
  fir_col_async6/15(real_out8) -> fir_col_async7/15(real8)
  fir_col_async6/14(imag_out7) -> fir_col_async7/14(imag7)
  fir_col_async6/13(real_out7) -> fir_col_async7/13(real7)
  fir_col_async6/12(imag_out6) -> fir_col_async7/12(imag6)
  fir_col_async6/11(real_out6) -> fir_col_async7/11(real6)
  fir_col_async6/10(imag_out5) -> fir_col_async7/10(imag5)
  fir_col_async6/9(real_out5) -> fir_col_async7/9(real5)
  fir_col_async6/8(imag_out4) -> fir_col_async7/8(imag4)
  fir_col_async6/7(real_out4) -> fir_col_async7/7(real4)
  fir_col_async6/6(imag_out3) -> fir_col_async7/6(imag3)
  fir_col_async6/5(real_out3) -> fir_col_async7/5(real3)
  fir_col_async6/4(imag_out2) -> fir_col_async7/4(imag2)
  fir_col_async6/3(real_out2) -> fir_col_async7/3(real2)
  fir_col_async6/2(imag_out1) -> fir_col_async7/2(imag1)
  fir_col_async6/1(real_out1) -> fir_col_async7/1(real1)
  fir_col_async6/66(imag_sum) -> imag_sum/7(din6)
  fir_col_async6/65(real_sum) -> real_sum/7(din6)
  fir_col_async5/32(imag_out16) -> fir_col_async6/32(imag16)
  fir_col_async5/31(real_out16) -> fir_col_async6/31(real16)
  fir_col_async5/30(imag_out15) -> fir_col_async6/30(imag15)
  fir_col_async5/29(real_out15) -> fir_col_async6/29(real15)
  fir_col_async5/28(imag_out14) -> fir_col_async6/28(imag14)
  fir_col_async5/27(real_out14) -> fir_col_async6/27(real14)
  fir_col_async5/26(imag_out13) -> fir_col_async6/26(imag13)
  fir_col_async5/25(real_out13) -> fir_col_async6/25(real13)
  fir_col_async5/24(imag_out12) -> fir_col_async6/24(imag12)
  fir_col_async5/23(real_out12) -> fir_col_async6/23(real12)
  fir_col_async5/22(imag_out11) -> fir_col_async6/22(imag11)
  fir_col_async5/21(real_out11) -> fir_col_async6/21(real11)
  fir_col_async5/20(imag_out10) -> fir_col_async6/20(imag10)
  fir_col_async5/19(real_out10) -> fir_col_async6/19(real10)
  fir_col_async5/18(imag_out9) -> fir_col_async6/18(imag9)
  fir_col_async5/17(real_out9) -> fir_col_async6/17(real9)
  fir_col_async5/16(imag_out8) -> fir_col_async6/16(imag8)
  fir_col_async5/15(real_out8) -> fir_col_async6/15(real8)
  fir_col_async5/14(imag_out7) -> fir_col_async6/14(imag7)
  fir_col_async5/13(real_out7) -> fir_col_async6/13(real7)
  fir_col_async5/12(imag_out6) -> fir_col_async6/12(imag6)
  fir_col_async5/11(real_out6) -> fir_col_async6/11(real6)
  fir_col_async5/10(imag_out5) -> fir_col_async6/10(imag5)
  fir_col_async5/9(real_out5) -> fir_col_async6/9(real5)
  fir_col_async5/8(imag_out4) -> fir_col_async6/8(imag4)
  fir_col_async5/7(real_out4) -> fir_col_async6/7(real4)
  fir_col_async5/6(imag_out3) -> fir_col_async6/6(imag3)
  fir_col_async5/5(real_out3) -> fir_col_async6/5(real3)
  fir_col_async5/4(imag_out2) -> fir_col_async6/4(imag2)
  fir_col_async5/3(real_out2) -> fir_col_async6/3(real2)
  fir_col_async5/2(imag_out1) -> fir_col_async6/2(imag1)
  fir_col_async5/1(real_out1) -> fir_col_async6/1(real1)
  fir_col_async5/66(imag_sum) -> imag_sum/6(din5)
  fir_col_async5/65(real_sum) -> real_sum/6(din5)
  fir_col_async4/32(imag_out16) -> fir_col_async5/32(imag16)
  fir_col_async4/31(real_out16) -> fir_col_async5/31(real16)
  fir_col_async4/30(imag_out15) -> fir_col_async5/30(imag15)
  fir_col_async4/29(real_out15) -> fir_col_async5/29(real15)
  fir_col_async4/28(imag_out14) -> fir_col_async5/28(imag14)
  fir_col_async4/27(real_out14) -> fir_col_async5/27(real14)
  fir_col_async4/26(imag_out13) -> fir_col_async5/26(imag13)
  fir_col_async4/25(real_out13) -> fir_col_async5/25(real13)
  fir_col_async4/24(imag_out12) -> fir_col_async5/24(imag12)
  fir_col_async4/23(real_out12) -> fir_col_async5/23(real12)
  fir_col_async4/22(imag_out11) -> fir_col_async5/22(imag11)
  fir_col_async4/21(real_out11) -> fir_col_async5/21(real11)
  fir_col_async4/20(imag_out10) -> fir_col_async5/20(imag10)
  fir_col_async4/19(real_out10) -> fir_col_async5/19(real10)
  fir_col_async4/18(imag_out9) -> fir_col_async5/18(imag9)
  fir_col_async4/17(real_out9) -> fir_col_async5/17(real9)
  fir_col_async4/16(imag_out8) -> fir_col_async5/16(imag8)
  fir_col_async4/15(real_out8) -> fir_col_async5/15(real8)
  fir_col_async4/14(imag_out7) -> fir_col_async5/14(imag7)
  fir_col_async4/13(real_out7) -> fir_col_async5/13(real7)
  fir_col_async4/12(imag_out6) -> fir_col_async5/12(imag6)
  fir_col_async4/11(real_out6) -> fir_col_async5/11(real6)
  fir_col_async4/10(imag_out5) -> fir_col_async5/10(imag5)
  fir_col_async4/9(real_out5) -> fir_col_async5/9(real5)
  fir_col_async4/8(imag_out4) -> fir_col_async5/8(imag4)
  fir_col_async4/7(real_out4) -> fir_col_async5/7(real4)
  fir_col_async4/6(imag_out3) -> fir_col_async5/6(imag3)
  fir_col_async4/5(real_out3) -> fir_col_async5/5(real3)
  fir_col_async4/4(imag_out2) -> fir_col_async5/4(imag2)
  fir_col_async4/3(real_out2) -> fir_col_async5/3(real2)
  fir_col_async4/2(imag_out1) -> fir_col_async5/2(imag1)
  fir_col_async4/1(real_out1) -> fir_col_async5/1(real1)
  fir_col_async4/66(imag_sum) -> imag_sum/5(din4)
  fir_col_async4/65(real_sum) -> real_sum/5(din4)
  fir_col_async3/32(imag_out16) -> fir_col_async4/32(imag16)
  fir_col_async3/31(real_out16) -> fir_col_async4/31(real16)
  fir_col_async3/30(imag_out15) -> fir_col_async4/30(imag15)
  fir_col_async3/29(real_out15) -> fir_col_async4/29(real15)
  fir_col_async3/28(imag_out14) -> fir_col_async4/28(imag14)
  fir_col_async3/27(real_out14) -> fir_col_async4/27(real14)
  fir_col_async3/26(imag_out13) -> fir_col_async4/26(imag13)
  fir_col_async3/25(real_out13) -> fir_col_async4/25(real13)
  fir_col_async3/24(imag_out12) -> fir_col_async4/24(imag12)
  fir_col_async3/23(real_out12) -> fir_col_async4/23(real12)
  fir_col_async3/22(imag_out11) -> fir_col_async4/22(imag11)
  fir_col_async3/21(real_out11) -> fir_col_async4/21(real11)
  fir_col_async3/20(imag_out10) -> fir_col_async4/20(imag10)
  fir_col_async3/19(real_out10) -> fir_col_async4/19(real10)
  fir_col_async3/18(imag_out9) -> fir_col_async4/18(imag9)
  fir_col_async3/17(real_out9) -> fir_col_async4/17(real9)
  fir_col_async3/16(imag_out8) -> fir_col_async4/16(imag8)
  fir_col_async3/15(real_out8) -> fir_col_async4/15(real8)
  fir_col_async3/14(imag_out7) -> fir_col_async4/14(imag7)
  fir_col_async3/13(real_out7) -> fir_col_async4/13(real7)
  fir_col_async3/12(imag_out6) -> fir_col_async4/12(imag6)
  fir_col_async3/11(real_out6) -> fir_col_async4/11(real6)
  fir_col_async3/10(imag_out5) -> fir_col_async4/10(imag5)
  fir_col_async3/9(real_out5) -> fir_col_async4/9(real5)
  fir_col_async3/8(imag_out4) -> fir_col_async4/8(imag4)
  fir_col_async3/7(real_out4) -> fir_col_async4/7(real4)
  fir_col_async3/6(imag_out3) -> fir_col_async4/6(imag3)
  fir_col_async3/5(real_out3) -> fir_col_async4/5(real3)
  fir_col_async3/4(imag_out2) -> fir_col_async4/4(imag2)
  fir_col_async3/3(real_out2) -> fir_col_async4/3(real2)
  fir_col_async3/2(imag_out1) -> fir_col_async4/2(imag1)
  fir_col_async3/1(real_out1) -> fir_col_async4/1(real1)
  fir_col_async3/66(imag_sum) -> imag_sum/4(din3)
  fir_col_async3/65(real_sum) -> real_sum/4(din3)
  fir_col_async2/32(imag_out16) -> fir_col_async3/32(imag16)
  fir_col_async2/31(real_out16) -> fir_col_async3/31(real16)
  fir_col_async2/30(imag_out15) -> fir_col_async3/30(imag15)
  fir_col_async2/29(real_out15) -> fir_col_async3/29(real15)
  fir_col_async2/28(imag_out14) -> fir_col_async3/28(imag14)
  fir_col_async2/27(real_out14) -> fir_col_async3/27(real14)
  fir_col_async2/26(imag_out13) -> fir_col_async3/26(imag13)
  fir_col_async2/25(real_out13) -> fir_col_async3/25(real13)
  fir_col_async2/24(imag_out12) -> fir_col_async3/24(imag12)
  fir_col_async2/23(real_out12) -> fir_col_async3/23(real12)
  fir_col_async2/22(imag_out11) -> fir_col_async3/22(imag11)
  fir_col_async2/21(real_out11) -> fir_col_async3/21(real11)
  fir_col_async2/20(imag_out10) -> fir_col_async3/20(imag10)
  fir_col_async2/19(real_out10) -> fir_col_async3/19(real10)
  fir_col_async2/18(imag_out9) -> fir_col_async3/18(imag9)
  fir_col_async2/17(real_out9) -> fir_col_async3/17(real9)
  fir_col_async2/16(imag_out8) -> fir_col_async3/16(imag8)
  fir_col_async2/15(real_out8) -> fir_col_async3/15(real8)
  fir_col_async2/14(imag_out7) -> fir_col_async3/14(imag7)
  fir_col_async2/13(real_out7) -> fir_col_async3/13(real7)
  fir_col_async2/12(imag_out6) -> fir_col_async3/12(imag6)
  fir_col_async2/11(real_out6) -> fir_col_async3/11(real6)
  fir_col_async2/10(imag_out5) -> fir_col_async3/10(imag5)
  fir_col_async2/9(real_out5) -> fir_col_async3/9(real5)
  fir_col_async2/8(imag_out4) -> fir_col_async3/8(imag4)
  fir_col_async2/7(real_out4) -> fir_col_async3/7(real4)
  fir_col_async2/6(imag_out3) -> fir_col_async3/6(imag3)
  fir_col_async2/5(real_out3) -> fir_col_async3/5(real3)
  fir_col_async2/4(imag_out2) -> fir_col_async3/4(imag2)
  fir_col_async2/3(real_out2) -> fir_col_async3/3(real2)
  fir_col_async2/2(imag_out1) -> fir_col_async3/2(imag1)
  fir_col_async2/1(real_out1) -> fir_col_async3/1(real1)
  fir_col_async2/66(imag_sum) -> imag_sum/3(din2)
  fir_col_async2/65(real_sum) -> real_sum/3(din2)
  fir_col_async1/32(imag_out16) -> fir_col_async2/32(imag16)
  fir_col_async1/31(real_out16) -> fir_col_async2/31(real16)
  fir_col_async1/30(imag_out15) -> fir_col_async2/30(imag15)
  fir_col_async1/29(real_out15) -> fir_col_async2/29(real15)
  fir_col_async1/28(imag_out14) -> fir_col_async2/28(imag14)
  fir_col_async1/27(real_out14) -> fir_col_async2/27(real14)
  fir_col_async1/26(imag_out13) -> fir_col_async2/26(imag13)
  fir_col_async1/25(real_out13) -> fir_col_async2/25(real13)
  fir_col_async1/24(imag_out12) -> fir_col_async2/24(imag12)
  fir_col_async1/23(real_out12) -> fir_col_async2/23(real12)
  fir_col_async1/22(imag_out11) -> fir_col_async2/22(imag11)
  fir_col_async1/21(real_out11) -> fir_col_async2/21(real11)
  fir_col_async1/20(imag_out10) -> fir_col_async2/20(imag10)
  fir_col_async1/19(real_out10) -> fir_col_async2/19(real10)
  fir_col_async1/18(imag_out9) -> fir_col_async2/18(imag9)
  fir_col_async1/17(real_out9) -> fir_col_async2/17(real9)
  fir_col_async1/16(imag_out8) -> fir_col_async2/16(imag8)
  fir_col_async1/15(real_out8) -> fir_col_async2/15(real8)
  fir_col_async1/14(imag_out7) -> fir_col_async2/14(imag7)
  fir_col_async1/13(real_out7) -> fir_col_async2/13(real7)
  fir_col_async1/12(imag_out6) -> fir_col_async2/12(imag6)
  fir_col_async1/11(real_out6) -> fir_col_async2/11(real6)
  fir_col_async1/10(imag_out5) -> fir_col_async2/10(imag5)
  fir_col_async1/9(real_out5) -> fir_col_async2/9(real5)
  fir_col_async1/8(imag_out4) -> fir_col_async2/8(imag4)
  fir_col_async1/7(real_out4) -> fir_col_async2/7(real4)
  fir_col_async1/6(imag_out3) -> fir_col_async2/6(imag3)
  fir_col_async1/5(real_out3) -> fir_col_async2/5(real3)
  fir_col_async1/4(imag_out2) -> fir_col_async2/4(imag2)
  fir_col_async1/3(real_out2) -> fir_col_async2/3(real2)
  fir_col_async1/2(imag_out1) -> fir_col_async2/2(imag1)
  fir_col_async1/1(real_out1) -> fir_col_async2/1(real1)
  fir_col_async1/66(imag_sum) -> imag_sum/2(din1)
  fir_col_async1/65(real_sum) -> real_sum/2(din1)
  imag16/1 -> fir_col_async1/32(imag16)
  real16/1 -> fir_col_async1/31(real16)
  imag15/1 -> fir_col_async1/30(imag15)
  real15/1 -> fir_col_async1/29(real15)
  imag14/1 -> fir_col_async1/28(imag14)
  real14/1 -> fir_col_async1/27(real14)
  imag13/1 -> fir_col_async1/26(imag13)
  real13/1 -> fir_col_async1/25(real13)
  imag12/1 -> fir_col_async1/24(imag12)
  real12/1 -> fir_col_async1/23(real12)
  imag11/1 -> fir_col_async1/22(imag11)
  real11/1 -> fir_col_async1/21(real11)
  imag10/1 -> fir_col_async1/20(imag10)
  real10/1 -> fir_col_async1/19(real10)
  imag9/1 -> fir_col_async1/18(imag9)
  real9/1 -> fir_col_async1/17(real9)
  imag8/1 -> fir_col_async1/16(imag8)
  real8/1 -> fir_col_async1/15(real8)
  imag7/1 -> fir_col_async1/14(imag7)
  real7/1 -> fir_col_async1/13(real7)
  imag6/1 -> fir_col_async1/12(imag6)
  real6/1 -> fir_col_async1/11(real6)
  imag5/1 -> fir_col_async1/10(imag5)
  real5/1 -> fir_col_async1/9(real5)
  imag4/1 -> fir_col_async1/8(imag4)
  real4/1 -> fir_col_async1/7(real4)
  imag3/1 -> fir_col_async1/6(imag3)
  real3/1 -> fir_col_async1/5(real3)
  imag2/1 -> fir_col_async1/4(imag2)
  real2/1 -> fir_col_async1/3(real2)
  imag1/1 -> fir_col_async1/2(imag1)
  real1/1 -> fir_col_async1/1(real1)
  dv_delay/1 -> dv_out/1
  dv_in/1 -> fir_col_async8/65(dv), fir_col_async7/65(dv), fir_col_async6/65(dv), fir_col_async5/65(dv), fir_col_async4/65(dv), fir_col_async3/65(dv), fir_col_async2/65(dv), fir_col_async1/65(dv), dv_delay/1
  sync_in/1 -> sync_delay/1
